simulink model "F90_XMED_02"  (R2025a)
settings: Solver=daessc  StartTime=0.0  StopTime=6  MaxStep=0.6  RelTol=1e-3  AbsTol=1e-3
InitFcn:
  | assert(evalin('base','exist(''target_map_initial_mmHg'',''var'')')==1,'F90:XMED02:MissingPublicInput','Missing target_map_initial_mmHg.');assert(evalin('base','exist(''target_map_final_mmHg'',''var'')')==1,'F90:XMED02:MissingPublicInput','Missing target_map_final_mmHg.');assert(evalin('base','exist(''target_step_time_s'',''var'')')==1,'F90:XMED02:MissingPublicInput','Missing target_step_time_s.');assert(evalin('base','exist(''systemic_resistance_scale'',''var'')')==1,'F90:XMED02:MissingPublicInput','Missing systemic_resistance_scale.');assert(evalin('base','exist(''heart_rate_bpm'',''var'')')==1,'F90:XMED02:MissingPublicInput','Missing heart_rate_bpm.');assert(evalin('base','exist(''pump_speed_limit_rpm'',''var'')')==1,'F90:XMED02:MissingPublicInput','Missing pump_speed_limit_rpm.');f90_mw=get_param(bdroot,'ModelWorkspace');f90_hr=evalin('base','heart_rate_bpm');assignin(f90_mw,'tc',1/(f90_hr/60));assignin(f90_mw,'ts',0.16+0.3/(f90_hr/60));assignin(f90_mw,'R3',evalin('base','systemic_resistance_scale'));assignin(f90_mw,'Tend',6);clear f90_mw f90_hr;
model workspace (MAT data in the model file):
  C1 = 0.22
  C2 = 1.46
  C3 = 20
  C4 = 0.09
  C5 = 2.67
  C6 = 46.7
  EdL = 0.1
  EdR = 0.03
  EsL = 1.375
  EsR = 0.328
  FwVolt = 1e-05
  L1 = 0.000825
  L2 = 0.0036
  L3 = 0.00075
  L4 = 0.00308
  OffCond = 1000
  PipL = 50
  PipR = 24
  R1 = 0.0037511
  R2 = 0.067501
  R3 = 1
  R3_fix = 1
  R3_nominal = 1
  R4 = 0.003751
  R5 = 0.003751
  R6 = 0.03376
  R7 = 0.101
  R8 = 0.003751
  RL = 0.08
  RPM_Setting = 0
  RR = 0.0175
  RmL = 0.08
  RmR = 0.0175
  SetHartRate = 155
  Tend = 6
  WaitTime = 0.022
  X10 = 71.112
  X100 = 23.836
  X110 = 11.294
  X120 = 112.76
  X20 = 8.88
  X30 = 70.516
  X40 = 67.337
  X50 = 3.328
  X60 = 105.52
  X70 = 13.417
  X80 = 0.786
  X90 = 13.393
  capSerRes = 1e-09
  onRes = 0.0001
  tc = 0.8
  ts = 0.4
undefined symbols (not defined in the file): heart_rate_bpm, pump_speed_limit_rpm, systemic_resistance_scale, target_map_final_mmHg, target_map_initial_mmHg, target_step_time_s
libraries: fl_lib x68, nesl_utility x26, ee_lib x4, SignalEditorBlockLib x1
settings Model: Creator=mnord  LastModifiedBy=SimuVerity Contributors
settings SolverCC: ZeroCrossAlgorithm=Adaptive  AlgebraicLoopSolver=TrustRegion
settings DataIOCC: SignalLogging=off
settings DebuggingCC: MaxConsecutiveZCsMsg=warning  IgnoredZcDiagnostic=none  UnconnectedInputMsg=warning  UnconnectedOutputMsg=warning  UnconnectedLineMsg=warning  SymbolicDimsDataTypeCodeGenerationDiagnostic=none
settings ModelReferenceCC: EnableRefExpFcnMdlSchedulingChecks=on
settings SFSimCC: CustomCodeUndefinedFunction=UseInterfaceOnly
settings RTWCC: GPUComputeCapability=3.5  DLArmComputeVersion=19.05
settings SimscapeCC: SimscapeLogSimulationStatistics=on  SimscapeLogDataHistory=10000.0

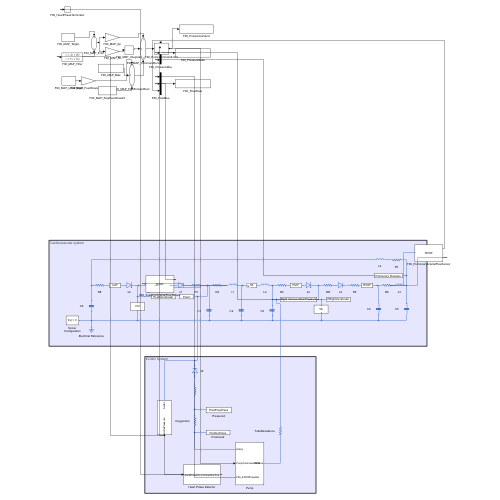
[thumbnail: Simulink's stored preview of the top-level diagram]
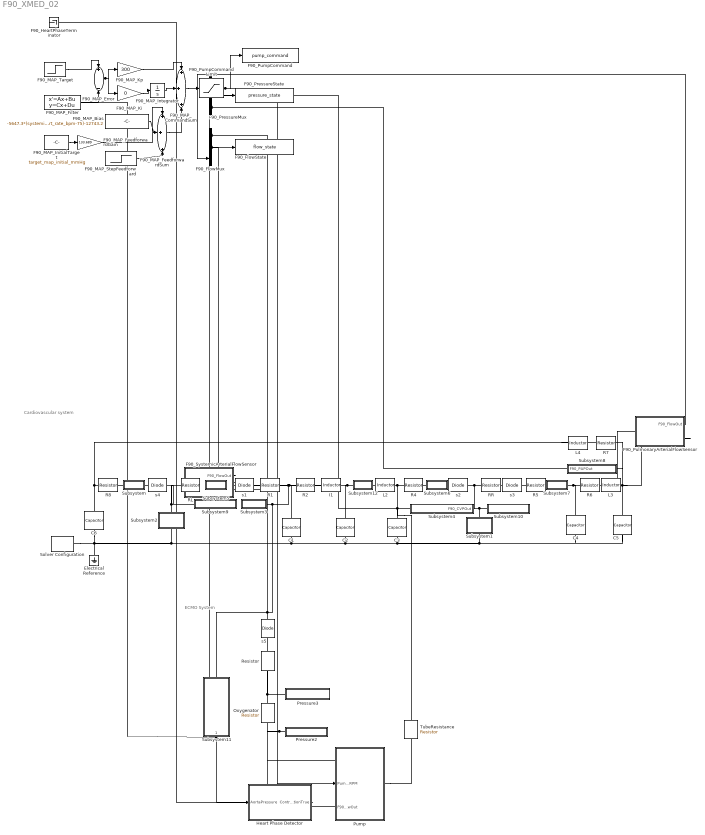
== system F90_XMED_02 ==
  note: Cardiovascular system
  note: ECMO System
  C1 : fl_lib/Electrical/Electrical Elements/Capacitor  c=C1 F  r=capSerRes Ohm  g=0 1/Ohm  i_specify=off  i_priority=None  i=0 A  i_nominal_specify=off  i_nominal_value=1  i_nominal_unit=A  v_specify=off  v_priority=High  v=X10 V  v_nominal_specify=off  v_nominal_value=1  v_nominal_unit=V  vc_specify=on  vc_priority=High  vc=X10 V  vc_nominal_specify=off  vc_nominal_value=1  vc_nominal_unit=V
  C2 : fl_lib/Electrical/Electrical Elements/Capacitor  c=C2 F  r=capSerRes Ohm  g=0 1/Ohm  i_specify=off  i_priority=None  i=0 A  i_nominal_specify=off  i_nominal_value=1  i_nominal_unit=A  v_specify=off  v_priority=High  v=X30 V  v_nominal_specify=off  v_nominal_value=1  v_nominal_unit=V  vc_specify=on  vc_priority=High  vc=X30 V  vc_nominal_specify=off  vc_nominal_value=1  vc_nominal_unit=V
  C3 : fl_lib/Electrical/Electrical Elements/Capacitor  c=C3 F  r=capSerRes Ohm  g=0 1/Ohm  i_specify=off  i_priority=None  i=0 A  i_nominal_specify=off  i_nominal_value=1  i_nominal_unit=A  v_specify=off  v_priority=High  v=X50 V  v_nominal_specify=off  v_nominal_value=1  v_nominal_unit=V  vc_specify=on  vc_priority=High  vc=X50 V  vc_nominal_specify=off  vc_nominal_value=1  vc_nominal_unit=V
  C4 : fl_lib/Electrical/Electrical Elements/Capacitor  c=C4 F  r=capSerRes Ohm  g=0 1/Ohm  i_specify=off  i_priority=None  i=0 A  i_nominal_specify=off  i_nominal_value=1  i_nominal_unit=A  v_specify=off  v_priority=High  v=X70 V  v_nominal_specify=off  v_nominal_value=1  v_nominal_unit=V  vc_specify=on  vc_priority=High  vc=X70 V  vc_nominal_specify=off  vc_nominal_value=1  vc_nominal_unit=V
  C5 : fl_lib/Electrical/Electrical Elements/Capacitor  c=C5 F  r=capSerRes Ohm  g=0 1/Ohm  i_specify=off  i_priority=None  i=0 A  i_nominal_specify=off  i_nominal_value=1  i_nominal_unit=A  v_specify=off  v_priority=High  v=X90 V  v_nominal_specify=off  v_nominal_value=1  v_nominal_unit=V  vc_specify=on  vc_priority=High  vc=X90 V  vc_nominal_specify=off  vc_nominal_value=1  vc_nominal_unit=V
  C6 : fl_lib/Electrical/Electrical Elements/Capacitor  c=C6 F  r=capSerRes Ohm  g=0 1/Ohm  i_specify=off  i_priority=None  i=0 A  i_nominal_specify=off  i_nominal_value=1  i_nominal_unit=A  v_specify=off  v_priority=High  v=X110 V  v_nominal_specify=off  v_nominal_value=1  v_nominal_unit=V  vc_specify=on  vc_priority=High  vc=X110 V  vc_nominal_specify=off  vc_nominal_value=1  vc_nominal_unit=V
  Electrical Reference : fl_lib/Electrical/Electrical Elements/Electrical Reference
  F90_FlowMux : Mux  Inputs=3
  F90_FlowState : ToWorkspace  VariableName=flow_state  SaveFormat=Timeseries  SampleTime=-1
  F90_HeartPhaseTerminator : Terminator
  F90_MAP_Bias : Constant  Value=-5647.3*(systemic_resistance_scale-1)-6.178*(heart_rate_bpm-75)-12743.2
  F90_MAP_CommandSum : Sum  Inputs=+++
  F90_MAP_Error : Sum  Inputs=+-
  F90_MAP_FeedforwardGain : Gain  Gain=133.689
  F90_MAP_FeedforwardSum : Sum  Inputs=+++
  F90_MAP_Filter : StateSpace  A=-1/0.35  B=1/0.35  D=0  InitialCondition=target_map_initial_mmHg
  F90_MAP_InitialTarget : Constant  Value=target_map_initial_mmHg
  F90_MAP_Integrator : Integrator
  F90_MAP_Ki : Gain  Gain=0
  F90_MAP_Kp : Gain  Gain=300
  F90_MAP_StepFeedforward : Step  Time=target_step_time_s  After=90*(target_map_final_mmHg-target_map_initial_mmHg)  SampleTime=0
  F90_MAP_Target : Step  Time=target_step_time_s  Before=target_map_initial_mmHg  After=target_map_final_mmHg  SampleTime=0
  F90_PressureMux : Mux  Inputs=3
  F90_PressureState : ToWorkspace  VariableName=pressure_state  SaveFormat=Timeseries  SampleTime=-1
  F90_PulmonaryArterialFlowSensor : Subsystem
      mask Display: disp('RVOF')
  F90_PumpCommand : ToWorkspace  VariableName=pump_command  SaveFormat=Timeseries  SampleTime=-1
  F90_PumpCommandLimit : Saturate  UpperLimit=pump_speed_limit_rpm  LowerLimit=0
  F90_SystemicArterialFlowSensor : Subsystem
      mask Display: disp('RVOF')
  Heart Phase Detector : Subsystem
  I1 : ee_lib/Passive/Inductor  l=L1 H  enable_L_tol=0  L_tol=20  tol_distribution=1  nSigma=4  r=0 Ohm  g=1e-9 1/Ohm  enable_operating_limits=0  operating_limit_action=2  max_working_current=1 A  power_rating=1 W  i_L_specify=on  i_L_priority=High  i_L=X20 A  i_L_nominal_specify=off  i_L_nominal_value=1  i_L_nominal_unit=A
  L2 : ee_lib/Passive/Inductor  l=L2 H  enable_L_tol=0  L_tol=20  tol_distribution=1  nSigma=4  r=0 Ohm  g=1e-9 1/Ohm  enable_operating_limits=0  operating_limit_action=2  max_working_current=1 A  power_rating=1 W  i_L_specify=on  i_L_priority=High  i_L=X40 A  i_L_nominal_specify=off  i_L_nominal_value=1  i_L_nominal_unit=A
  L3 : ee_lib/Passive/Inductor  l=L3 H  enable_L_tol=0  L_tol=20  tol_distribution=1  nSigma=4  r=0 Ohm  g=1e-9 1/Ohm  enable_operating_limits=0  operating_limit_action=2  max_working_current=1 A  power_rating=1 W  i_L_specify=on  i_L_priority=High  i_L=X80 A  i_L_nominal_specify=off  i_L_nominal_value=1  i_L_nominal_unit=A
  L4 : ee_lib/Passive/Inductor  l=L4 H  enable_L_tol=0  L_tol=20  tol_distribution=1  nSigma=4  r=0 Ohm  g=1e-9 1/Ohm  enable_operating_limits=0  operating_limit_action=2  max_working_current=1 A  power_rating=1 W  i_L_specify=on  i_L_priority=High  i_L=X100 A  i_L_nominal_specify=off  i_L_nominal_value=1  i_L_nominal_unit=A
  Oxygenator : fl_lib/Electrical/Electrical Elements/Resistor  R=1/1.13 Ohm  i_specify=off  i_priority=None  i=0 A  i_nominal_specify=off  i_nominal_value=1  i_nominal_unit=A  v_specify=off  v_priority=None  v=0 V  v_nominal_specify=off  v_nominal_value=1  v_nominal_unit=V
  Pressure2 : Subsystem
      mask Display: disp('PreOxyPress')
  Pressure3 : Subsystem
      mask Display: disp('PostPoxyPress')
  Pump : Subsystem
      settings: PortSchema="{\"entries\":[{\"content\":{\"sides\":[{\"content\":{\"connectorIds\":[\"LConn1\"]},\"type\":\"ConnectorPlacement.EquallySpacedRectSide\",\"uuid\":\"62db16dc-542a-4803-9c2c-9a470fc91885\"},{\"content\":{\"connectorIds\":[\"RConn1\",\"In1\",\"Out1\"],\"side\":\"RIGHT\"},\"type\":\"ConnectorPlacement.EquallySpacedRectSide\",\"uuid\":\"05a4665e-1cd6-4c93-95ba-f78495d840a1\"},{\"content\":{\"side\":\"TOP\"},\"type\":\"ConnectorPlacement.EquallySpacedRectSide\",\"uuid\":\"174192fa-e994-4b45-8a1f-dd44ebe2b866\"},{\"content\":{\"side\":\"BOTTOM\"},\"type\":\"ConnectorPlacement.EquallySpacedRectSide\",\"uuid\":\"194a326f-2a13-4189-b0b8-d4f935dc1fe6\"}]},\"type\":\"ConnectorPlacement.EquallySpacedConnector\",\"uuid\":\"9d7b36c7-1763-48ea-a53e-009c812e3b66\"}],\"packageUris\":[\"http://schema.mathworks.com/mf0/Connector/R2020b\"],\"version\":\"1.0\"}"
  R1 : fl_lib/Electrical/Electrical Elements/Resistor  R=R1 Ohm  i_specify=off  i_priority=None  i=0 A  i_nominal_specify=off  i_nominal_value=1  i_nominal_unit=A  v_specify=off  v_priority=None  v=0 V  v_nominal_specify=off  v_nominal_value=1  v_nominal_unit=V
  R2 : fl_lib/Electrical/Electrical Elements/Resistor  R=R2 Ohm  i_specify=off  i_priority=None  i=0 A  i_nominal_specify=off  i_nominal_value=1  i_nominal_unit=A  v_specify=off  v_priority=None  v=0 V  v_nominal_specify=off  v_nominal_value=1  v_nominal_unit=V
  R4 : fl_lib/Electrical/Electrical Elements/Resistor  R=R4 Ohm  i_specify=off  i_priority=None  i=0 A  i_nominal_specify=off  i_nominal_value=1  i_nominal_unit=A  v_specify=off  v_priority=None  v=0 V  v_nominal_specify=off  v_nominal_value=1  v_nominal_unit=V
  R5 : fl_lib/Electrical/Electrical Elements/Resistor  R=R5 Ohm  i_specify=off  i_priority=None  i=0 A  i_nominal_specify=off  i_nominal_value=1  i_nominal_unit=A  v_specify=off  v_priority=None  v=0 V  v_nominal_specify=off  v_nominal_value=1  v_nominal_unit=V
  R6 : fl_lib/Electrical/Electrical Elements/Resistor  R=R6 Ohm  i_specify=off  i_priority=None  i=0 A  i_nominal_specify=off  i_nominal_value=1  i_nominal_unit=A  v_specify=off  v_priority=None  v=0 V  v_nominal_specify=off  v_nominal_value=1  v_nominal_unit=V
  R7 : fl_lib/Electrical/Electrical Elements/Resistor  R=R7 Ohm  i_specify=off  i_priority=None  i=0 A  i_nominal_specify=off  i_nominal_value=1  i_nominal_unit=A  v_specify=off  v_priority=None  v=0 V  v_nominal_specify=off  v_nominal_value=1  v_nominal_unit=V
  R8 : fl_lib/Electrical/Electrical Elements/Resistor  R=R8 Ohm  i_specify=off  i_priority=None  i=0 A  i_nominal_specify=off  i_nominal_value=1  i_nominal_unit=A  v_specify=off  v_priority=None  v=0 V  v_nominal_specify=off  v_nominal_value=1  v_nominal_unit=V
  RL : fl_lib/Electrical/Electrical Elements/Resistor  R=RL Ohm  i_specify=off  i_priority=None  i=0 A  i_nominal_specify=off  i_nominal_value=1  i_nominal_unit=A  v_specify=off  v_priority=None  v=0 V  v_nominal_specify=off  v_nominal_value=1  v_nominal_unit=V
  RR : fl_lib/Electrical/Electrical Elements/Resistor  R=RR Ohm  i_specify=off  i_priority=None  i=0 A  i_nominal_specify=off  i_nominal_value=1  i_nominal_unit=A  v_specify=off  v_priority=None  v=0 V  v_nominal_specify=off  v_nominal_value=1  v_nominal_unit=V
  Resistor : fl_lib/Electrical/Electrical Elements/Resistor  R=1/1.6 Ohm  i_specify=off  i_priority=None  i=0 A  i_nominal_specify=off  i_nominal_value=1  i_nominal_unit=A  v_specify=off  v_priority=None  v=0 V  v_nominal_specify=off  v_nominal_value=1  v_nominal_unit=V
  Solver Configuration : nesl_utility/Solver Configuration  PhysicalDomain=network_engine_domain  SubClassName=solver  LeftPortType=input  RightPortType=generic  Tones=[]  Harmonics=[]  SimulateNoise=off  Profile=off  UseLocalSampling=off  EnableSwitchedLinearOptims=on  FrequencyDomain=off  UseCCode=off  RelTol=0.001  AbsTol=1e-06  MinStep=1e-09  ToWorkspace=off  RevertToSquareIcSolve=off  NumHomotopyIterations=100  PhasorMode=off  PhasorModeNumHarmonics=1  ConsistencySolver=NEWTON_FTOL  IndexReductionMethod=DerivativeReplacement  DoDC=off  ResidualTolerance=1e-09  ConsistencyTolSource=GLOBAL  ConsistencyAbsTol=0.001  ConsistencyRelTol=0.001  ConsistencyTolFactor=0.001  UseLocalSolver=off  LocalSolverChoice=NE_BACKWARD_EULER_ADVANCER  ResolveIndetEquations=on  FunctionEvalNumThread=1  LocalSolverSampleTime=0.001  DoFixedCost=off  MaxNonlinIter=3  MaxModeIter=2  ComputeImpulses=off  ImpulseIterations=2  LinearAlgebra=auto  LinearAlgebraNumThread=0  EquationFormulation=NE_TIME_EF  DelaysMemoryBudget=1024  AutomaticFiltering=on  FilteringTimeConstant=0.001  PartitionStorageMethod=AS_NEEDED  PartitionMemoryBudget=1024  PartitionMethod=ROBUST  MultibodyUseLocalSolver=off  MultibodyLocalSolverChoice=ODE1  MultibodyLocalSolverSampleTime=0.001
  Subsystem : Subsystem
      mask Display: disp('LVIF')
  Subsystem1 : Subsystem
      mask Display: disp('V6')
  Subsystem10 : Subsystem
      mask Display: disp('PRightVentricular')
  Subsystem11 : Subsystem
      settings: PortSchema="{\"entries\":[{\"content\":{\"sides\":[{\"content\":{\"connectorIds\":[]},\"type\":\"ConnectorPlacement.EquallySpacedRectSide\",\"uuid\":\"f9ffc3b3-0f3f-4df5-be7e-a65199d8fb18\"},{\"content\":{\"connectorIds\":[],\"side\":\"RIGHT\"},\"type\":\"ConnectorPlacement.EquallySpacedRectSide\",\"uuid\":\"6b3c46a3-b656-482e-b0a9-93777308e083\"},{\"content\":{\"connectorIds\":[\"LConn1\"],\"side\":\"TOP\"},\"type\":\"ConnectorPlacement.EquallySpacedRectSide\",\"uuid\":\"e2309b6a-a528-4e82-8df5-2fdb2444f40a\"},{\"content\":{\"connectorIds\":[\"Out1\"],\"side\":\"BOTTOM\"},\"type\":\"ConnectorPlacement.EquallySpacedRectSide\",\"uuid\":\"7e89f23f-224f-485d-9e96-fb39bd2403a7\"}]},\"type\":\"ConnectorPlacement.EquallySpacedConnector\",\"uuid\":\"798f20cf-0f77-4082-bc02-f5f2bf5391c0\"}],\"packageUris\":[\"http://schema.mathworks.com/mf0/Connector/R2020b\"],\"version\":\"1.0\"}"
  Subsystem12 : Subsystem  Variant=on  VariantControlMode=label  VariantControl=Choice  LabelModeActiveChoice=R3_Fix
      mask Display: disp('R3')
  Subsystem2 : Subsystem
      mask Display: disp('V12')
  Subsystem3 : Subsystem
      mask Display: disp('Paort')
  Subsystem4 : Subsystem
      mask Display: disp('Right Venous Atrial Pressure')
  Subsystem5 : Subsystem
      mask Display: disp('LVOF')
  Subsystem6 : Subsystem
      mask Display: disp('RVIF')
  Subsystem7 : Subsystem
      mask Display: disp('RVOF')
  Subsystem8 : Subsystem
      mask Display: disp('Pulmonary Pressure')
  Subsystem9 : Subsystem
      mask Display: disp('PLeftVentricular')
  TubeResistance : fl_lib/Electrical/Electrical Elements/Resistor  R=1 Ohm  i_specify=off  i_priority=None  i=60 A  i_nominal_specify=off  i_nominal_value=1  i_nominal_unit=A  v_specify=off  v_priority=None  v=0 V  v_nominal_specify=off  v_nominal_value=1  v_nominal_unit=V
  s{1..4} (4 alike) : fl_lib/Electrical/Electrical Elements/Diode  Vf=FwVolt V  Ron=onRes Ohm  Goff=1e-8 1/Ohm  i_specify=off  i_priority=None  i=0 A  i_nominal_specify=off  i_nominal_value=1  i_nominal_unit=A  v_specify=off  v_priority=None  v=0 V  v_nominal_specify=off  v_nominal_value=1  v_nominal_unit=V
  s5 : fl_lib/Electrical/Electrical Elements/Diode  Vf=FwVolt V  Ron=0.54*0.1 Ohm  Goff=1e-8 1/Ohm  i_specify=off  i_priority=None  i=0 A  i_nominal_specify=off  i_nominal_value=1  i_nominal_unit=A  v_specify=off  v_priority=None  v=0 V  v_nominal_specify=off  v_nominal_value=1  v_nominal_unit=V
  wires:
  Subsystem11/1(AortaPressure) -> Heart Phase Detector/1(AortaPressure), F90_PressureMux/1, F90_MAP_Filter/1
  Heart Phase Detector/1(ContractionTrue) -> F90_HeartPhaseTerminator/1
  Subsystem4/1(F90_CVPOut) -> F90_PressureMux/2
  Subsystem8/1(F90_PAPOut) -> F90_PressureMux/3
  F90_PressureMux/1 -> F90_PressureState/1
  Pump/1(F90_ECMOFlowOut) -> F90_FlowMux/1
  F90_SystemicArterialFlowSensor/1(F90_FlowOut) -> F90_FlowMux/2
  F90_PulmonaryArterialFlowSensor/1(F90_FlowOut) -> F90_FlowMux/3
  F90_FlowMux/1 -> F90_FlowState/1
  F90_MAP_Target/1 -> F90_MAP_Error/1
  F90_MAP_Filter/1 -> F90_MAP_Error/2
  F90_MAP_Error/1 -> F90_MAP_Kp/1, F90_MAP_Ki/1
  F90_MAP_Kp/1 -> F90_MAP_CommandSum/1
  F90_MAP_Ki/1 -> F90_MAP_Integrator/1
  F90_MAP_Integrator/1 -> F90_MAP_CommandSum/2
  F90_MAP_InitialTarget/1 -> F90_MAP_FeedforwardGain/1
  F90_MAP_FeedforwardGain/1 -> F90_MAP_FeedforwardSum/1
  F90_MAP_Bias/1 -> F90_MAP_FeedforwardSum/2
  F90_MAP_StepFeedforward/1 -> F90_MAP_FeedforwardSum/3
  F90_MAP_FeedforwardSum/1 -> F90_MAP_CommandSum/3
  F90_MAP_CommandSum/1 -> F90_PumpCommandLimit/1
  F90_PumpCommandLimit/1 -> Pump/1(PumpCommandRPM), F90_PumpCommand/1
  connections:
  s1/LConn1 -- Subsystem5/RConn1
  s2/LConn1 -- Subsystem6/RConn1
  R5/RConn1 -- Subsystem7/LConn1
  s4/LConn1 -- Subsystem/RConn1
  R6/LConn1 -- C4/LConn1 -- Subsystem7/RConn1
  Subsystem12/RConn1 -- L2/LConn1
  Subsystem5/LConn1 -- RL/RConn1
  L3/RConn1 -- Subsystem8/LConn1 -- R7/LConn1 -- C5/LConn1
  Subsystem6/LConn1 -- R4/RConn1
  C6/LConn1 -- R8/LConn1 -- L4/RConn1
  s1/RConn1 -- R1/LConn1
  s3/RConn1 -- R5/LConn1
  R7/RConn1 -- L4/LConn1
  R8/RConn1 -- Subsystem/LConn1
  Subsystem10/LConn1 -- Subsystem1/LConn1 -- RR/LConn1 -- s2/RConn1
  s4/RConn1 -- RL/LConn1 -- Subsystem9/LConn1 -- Subsystem2/LConn1
  s3/LConn1 -- RR/RConn1
  C6/RConn1 -- Electrical Reference/LConn1 -- C5/RConn1 -- C4/RConn1 -- Subsystem1/RConn1 -- C3/RConn1 -- C2/RConn1 -- C1/RConn1 -- Subsystem2/RConn1 -- Solver Configuration/RConn1
  I1/RConn1 -- C2/LConn1 -- Subsystem12/LConn1
  Pressure2/RConn1 -- Pump/RConn1 -- Oxygenator/LConn1
  R4/LConn1 -- TubeResistance/LConn1 -- Subsystem4/LConn1 -- C3/LConn1 -- L2/RConn1
  Resistor/RConn1 -- s5/LConn1
  Oxygenator/RConn1 -- Resistor/LConn1 -- Pressure3/RConn1
  Pump/LConn1 -- TubeResistance/RConn1
  C1/LConn1 -- R1/RConn1 -- Subsystem11/LConn1 -- s5/RConn1 -- Subsystem3/LConn1 -- R2/LConn1
  R2/RConn1 -- F90_SystemicArterialFlowSensor/LConn1
  F90_SystemicArterialFlowSensor/RConn1 -- I1/LConn1
  R6/RConn1 -- F90_PulmonaryArterialFlowSensor/LConn1
  F90_PulmonaryArterialFlowSensor/RConn1 -- L3/LConn1

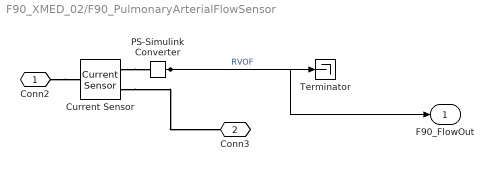
== system F90_XMED_02/F90_PulmonaryArterialFlowSensor ==
  Current Sensor : fl_lib/Electrical/Electrical Sensors/Current Sensor
  PS-Simulink Converter : nesl_utility/PS-Simulink Converter  PhysicalDomain=network_engine_domain  SubClassName=ps_output  LeftPortType=input  RightPortType=output  PseudoPeriodic=off  Frequencies=[]  VectorFormat=1-D array  Unit=inherit  AffineConversion=off
  Terminator : Terminator
  Conn2 : PMIOPort  Side=Left
  Conn3 : PMIOPort  Port=2  Side=Right
  F90_FlowOut : Outport
  wires:
  PS-Simulink Converter/1 -> Terminator/1, F90_FlowOut/1  "RVOF"
  connections:
  Current Sensor/RConn1 -- PS-Simulink Converter/LConn1
  Current Sensor/RConn2 -- Conn3/RConn1
  Conn2/RConn1 -- Current Sensor/LConn1

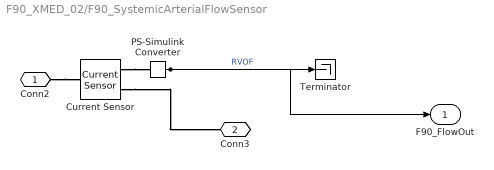
== system F90_XMED_02/F90_SystemicArterialFlowSensor ==
  Current Sensor : fl_lib/Electrical/Electrical Sensors/Current Sensor
  PS-Simulink Converter : nesl_utility/PS-Simulink Converter  PhysicalDomain=network_engine_domain  SubClassName=ps_output  LeftPortType=input  RightPortType=output  PseudoPeriodic=off  Frequencies=[]  VectorFormat=1-D array  Unit=inherit  AffineConversion=off
  Terminator : Terminator
  Conn2 : PMIOPort  Side=Left
  Conn3 : PMIOPort  Port=2  Side=Right
  F90_FlowOut : Outport
  wires:
  PS-Simulink Converter/1 -> Terminator/1, F90_FlowOut/1  "RVOF"
  connections:
  Current Sensor/RConn1 -- PS-Simulink Converter/LConn1
  Current Sensor/RConn2 -- Conn3/RConn1
  Conn2/RConn1 -- Current Sensor/LConn1

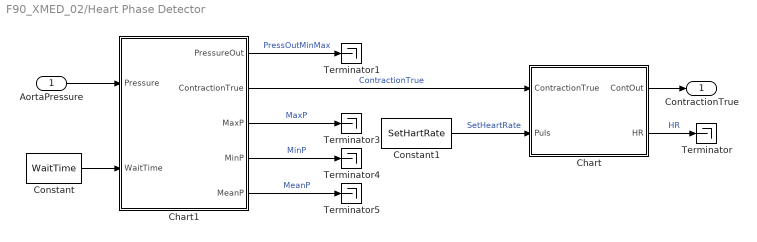
== system F90_XMED_02/Heart Phase Detector ==
  AortaPressure : Inport
  Chart : Stateflow chart  TreatAsAtomicUnit=on
  Chart1 : Stateflow chart  TreatAsAtomicUnit=on
  Constant : Constant  Value=WaitTime
  Constant1 : Constant  Value=SetHartRate
  Terminator{,1,3..5} (5 alike) : Terminator
  ContractionTrue : Outport
  wires:
  AortaPressure/1 -> Chart1/1(Pressure)
  Chart1/1(PressureOut) -> Terminator1/1  "PressOutMinMax"
  Chart1/2(ContractionTrue) -> Chart/1(ContractionTrue)  "ContractionTrue"
  Chart1/4(MinP) -> Terminator4/1  "MinP"
  Chart1/3(MaxP) -> Terminator3/1  "MaxP"
  Chart1/5(MeanP) -> Terminator5/1  "MeanP"
  Constant/1 -> Chart1/2(WaitTime)
  Chart/1(ContOut) -> ContractionTrue/1
  Chart/2(HR) -> Terminator/1  "HR"
  Constant1/1 -> Chart/2(Puls)  "SetHeartRate"

== system F90_XMED_02/Pressure2 ==
  Electrical Reference1 : fl_lib/Electrical/Electrical Elements/Electrical Reference
  Pre Oxy P2 : nesl_utility/PS-Simulink Converter  PhysicalDomain=network_engine_domain  SubClassName=ps_output  LeftPortType=input  RightPortType=output  PseudoPeriodic=off  Frequencies=[]  VectorFormat=1-D array  Unit=inherit  AffineConversion=off
  Pressure 2 : Scope
      settings: ActiveDisplayYMinimum=-9.53147  ActiveDisplayYMaximum=105.78415
  Voltage Sensor : fl_lib/Electrical/Electrical Sensors/Voltage Sensor
  Conn1 : PMIOPort  Side=Right
  wires:
  Pre Oxy P2/1 -> Pressure 2/1
  connections:
  Voltage Sensor/RConn1 -- Pre Oxy P2/LConn1
  Voltage Sensor/LConn1 -- Conn1/RConn1
  Voltage Sensor/RConn2 -- Electrical Reference1/LConn1

== system F90_XMED_02/Pressure3 ==
  Electrical Reference2 : fl_lib/Electrical/Electrical Elements/Electrical Reference
  Post Oxy P3 : nesl_utility/PS-Simulink Converter  PhysicalDomain=network_engine_domain  SubClassName=ps_output  LeftPortType=input  RightPortType=output  PseudoPeriodic=off  Frequencies=[]  VectorFormat=1-D array  Unit=inherit  AffineConversion=off
  Pressure3 : Scope
      settings: ActiveDisplayYMinimum=74.08538  ActiveDisplayYMaximum=102.93086
  Voltage Sensor : fl_lib/Electrical/Electrical Sensors/Voltage Sensor
  Conn1 : PMIOPort  Side=Right
  wires:
  Post Oxy P3/1 -> Pressure3/1
  connections:
  Voltage Sensor/RConn1 -- Post Oxy P3/LConn1
  Electrical Reference2/LConn1 -- Voltage Sensor/RConn2
  Conn1/RConn1 -- Voltage Sensor/LConn1

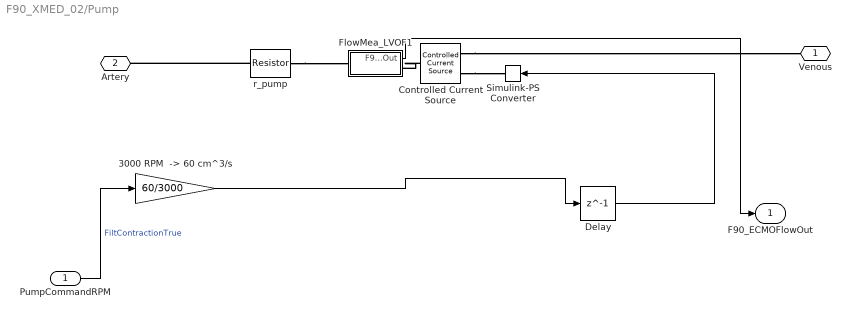
== system F90_XMED_02/Pump ==
  PumpCommandRPM : Inport
  "3000 RPM  -> 60 cm^3/s" : Gain  Gain=60/3000
  Controlled Current Source : fl_lib/Electrical/Electrical Sources/Controlled Current Source
  Delay : Delay  DelayLength=1  SampleTime=0.001
  FlowMea_LVOF1 : Subsystem
      mask Display: disp('EcmoFlow')
  Simulink-PS Converter : nesl_utility/Simulink-PS Converter  PhysicalDomain=network_engine_domain  SubClassName=ps_input  LeftPortType=input  RightPortType=output  PseudoPeriodic=off  Frequencies=[]  NoiseDistribution=none  NoiseParameters=[]  Unit=1  AffineConversion=off  FilteringAndDerivatives=filter  SimscapeFilterOrder=1  InputFilterTimeConstant=0.001  UdotUserProvided=0
  r_pump : fl_lib/Electrical/Electrical Elements/Resistor  R=1/1.68 Ohm  i_specify=on  i_priority=None  i=83.3 A  i_nominal_specify=off  i_nominal_value=1  i_nominal_unit=A  v_specify=off  v_priority=None  v=0 V  v_nominal_specify=off  v_nominal_value=1  v_nominal_unit=V
  Venous : PMIOPort  Side=Left
  Artery : PMIOPort  Port=2  Side=Right
  F90_ECMOFlowOut : Outport
  wires:
  Delay/1 -> Simulink-PS Converter/1
  PumpCommandRPM/1 -> "3000 RPM  -> 60 cm^3/s"/1  "FiltContractionTrue"
  "3000 RPM  -> 60 cm^3/s"/1 -> Delay/1
  FlowMea_LVOF1/1(F90_ECMOFlowOut) -> F90_ECMOFlowOut/1
  connections:
  Controlled Current Source/RConn2 -- Venous/RConn1
  r_pump/LConn1 -- FlowMea_LVOF1/LConn1
  Controlled Current Source/RConn1 -- Simulink-PS Converter/RConn1
  r_pump/RConn1 -- Artery/RConn1
  Controlled Current Source/LConn1 -- FlowMea_LVOF1/RConn1

== system F90_XMED_02/Subsystem ==
  Current Sensor : fl_lib/Electrical/Electrical Sensors/Current Sensor
  PS-Simulink Converter : nesl_utility/PS-Simulink Converter  PhysicalDomain=network_engine_domain  SubClassName=ps_output  LeftPortType=input  RightPortType=output  PseudoPeriodic=off  Frequencies=[]  VectorFormat=1-D array  Unit=inherit  AffineConversion=off
  Terminator : Terminator
  Conn2 : PMIOPort  Side=Left
  Conn3 : PMIOPort  Port=2  Side=Right
  wires:
  PS-Simulink Converter/1 -> Terminator/1  "LVIF"
  connections:
  Conn2/RConn1 -- Current Sensor/LConn1
  Current Sensor/RConn2 -- Conn3/RConn1
  Current Sensor/RConn1 -- PS-Simulink Converter/LConn1

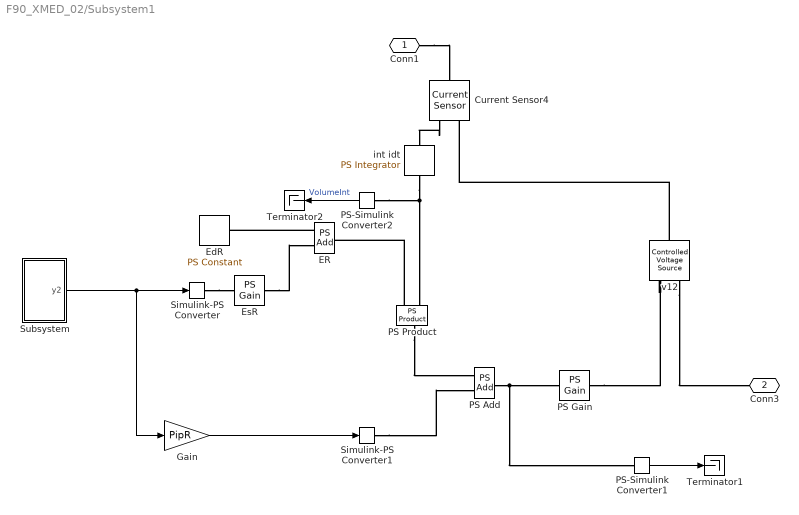
== system F90_XMED_02/Subsystem1 ==
  Current Sensor4 : fl_lib/Electrical/Electrical Sensors/Current Sensor
  ER : fl_lib/Physical Signals/Functions/PS Add
  EdR : fl_lib/Physical Signals/Sources/PS Constant  constant=EdR
  EsR : fl_lib/Physical Signals/Functions/PS Gain  gain=EsR
  Gain : Gain  Gain=PipR
  PS Add : fl_lib/Physical Signals/Functions/PS Add
  PS Gain : fl_lib/Physical Signals/Functions/PS Gain  gain=1 V/s/A
  PS Product : fl_lib/Physical Signals/Functions/PS Product
  PS-Simulink Converter1 : nesl_utility/PS-Simulink Converter  PhysicalDomain=network_engine_domain  SubClassName=ps_output  LeftPortType=input  RightPortType=output  PseudoPeriodic=off  Frequencies=[]  VectorFormat=1-D array  Unit=inherit  AffineConversion=off
  PS-Simulink Converter2 : nesl_utility/PS-Simulink Converter  PhysicalDomain=network_engine_domain  SubClassName=ps_output  LeftPortType=input  RightPortType=output  PseudoPeriodic=off  Frequencies=[]  VectorFormat=1-D array  Unit=inherit  AffineConversion=off
  Simulink-PS Converter : nesl_utility/Simulink-PS Converter  PhysicalDomain=network_engine_domain  SubClassName=ps_input  LeftPortType=input  RightPortType=output  PseudoPeriodic=off  Frequencies=[]  NoiseDistribution=none  NoiseParameters=[]  Unit=1  AffineConversion=off  FilteringAndDerivatives=provide  SimscapeFilterOrder=1  InputFilterTimeConstant=0.001  UdotUserProvided=0
  Simulink-PS Converter1 : nesl_utility/Simulink-PS Converter  PhysicalDomain=network_engine_domain  SubClassName=ps_input  LeftPortType=input  RightPortType=output  PseudoPeriodic=off  Frequencies=[]  NoiseDistribution=none  NoiseParameters=[]  Unit=A*s  AffineConversion=off  FilteringAndDerivatives=provide  SimscapeFilterOrder=1  InputFilterTimeConstant=0.001  UdotUserProvided=0
  Subsystem : Subsystem
  Terminator1 : Terminator
  Terminator2 : Terminator
  int idt : fl_lib/Physical Signals/Linear Operators/PS Integrator  reset_method=foundation.enum.IntegratorResetSpec.None  initial_condition_spec=foundation.enum.IntegratorICSpec.Internal  saturation_spec=foundation.enum.IntegratorSaturationSpec.None  saturation_source_spec=foundation.enum.IntegratorSaturationSourceSpec.Internal  x0=X60 A*s  xu=inf s  xl=-inf s
  v12 : fl_lib/Electrical/Electrical Sources/Controlled Voltage Source
  Conn1 : PMIOPort  Side=Left
  Conn3 : PMIOPort  Port=2  Side=Right
  wires:
  PS-Simulink Converter1/1 -> Terminator1/1
  Gain/1 -> Simulink-PS Converter1/1
  PS-Simulink Converter2/1 -> Terminator2/1  "VolumeInt"
  Subsystem/1(y2) -> Gain/1, Simulink-PS Converter/1
  connections:
  PS Add/RConn1 -- PS-Simulink Converter1/LConn1 -- PS Gain/LConn1
  PS-Simulink Converter2/LConn1 -- PS Product/LConn1 -- int idt/RConn1
  PS Product/RConn1 -- PS Add/LConn1
  v12/LConn1 -- Current Sensor4/RConn2
  ER/LConn1 -- EdR/RConn1
  Simulink-PS Converter1/RConn1 -- PS Add/LConn2
  EsR/RConn1 -- ER/LConn2
  PS Product/LConn2 -- ER/RConn1
  v12/RConn2 -- Conn3/RConn1
  Conn1/RConn1 -- Current Sensor4/LConn1
  Current Sensor4/RConn1 -- int idt/LConn1
  Simulink-PS Converter/RConn1 -- EsR/LConn1
  PS Gain/RConn1 -- v12/RConn1

== system F90_XMED_02/Subsystem10 ==
  Electrical Reference1 : fl_lib/Electrical/Electrical Elements/Electrical Reference
  PS-Simulink Converter : nesl_utility/PS-Simulink Converter  PhysicalDomain=network_engine_domain  SubClassName=ps_output  LeftPortType=input  RightPortType=output  PseudoPeriodic=off  Frequencies=[]  VectorFormat=1-D array  Unit=inherit  AffineConversion=off
  Terminator : Terminator
  Voltage Sensor : fl_lib/Electrical/Electrical Sensors/Voltage Sensor
  Conn1 : PMIOPort  Side=Left
  wires:
  PS-Simulink Converter/1 -> Terminator/1  "Right Ventricular Pressure"
  connections:
  Conn1/RConn1 -- Voltage Sensor/LConn1
  Voltage Sensor/RConn2 -- Electrical Reference1/LConn1
  Voltage Sensor/RConn1 -- PS-Simulink Converter/LConn1

== system F90_XMED_02/Subsystem11 ==
  Electrical Reference : fl_lib/Electrical/Electrical Elements/Electrical Reference
  PS-Simulink Converter : nesl_utility/PS-Simulink Converter  PhysicalDomain=network_engine_domain  SubClassName=ps_output  LeftPortType=input  RightPortType=output  PseudoPeriodic=off  Frequencies=[]  VectorFormat=1-D array  Unit=inherit  AffineConversion=off
  Voltage Sensor : fl_lib/Electrical/Electrical Sensors/Voltage Sensor
  Aorta1 : PMIOPort  Side=Left
  AortaPressure : Outport
  wires:
  PS-Simulink Converter/1 -> AortaPressure/1
  connections:
  Voltage Sensor/LConn1 -- Aorta1/RConn1
  Voltage Sensor/RConn2 -- Electrical Reference/LConn1
  Voltage Sensor/RConn1 -- PS-Simulink Converter/LConn1

== system F90_XMED_02/Subsystem12 ==
  Fixed : Subsystem  VariantControl=R3_Fix
  Variable : Subsystem  VariantControl=R3_Variant
  Conn1 : PMIOPort  Side=Left
  Conn2 : PMIOPort  Port=2  Side=Right

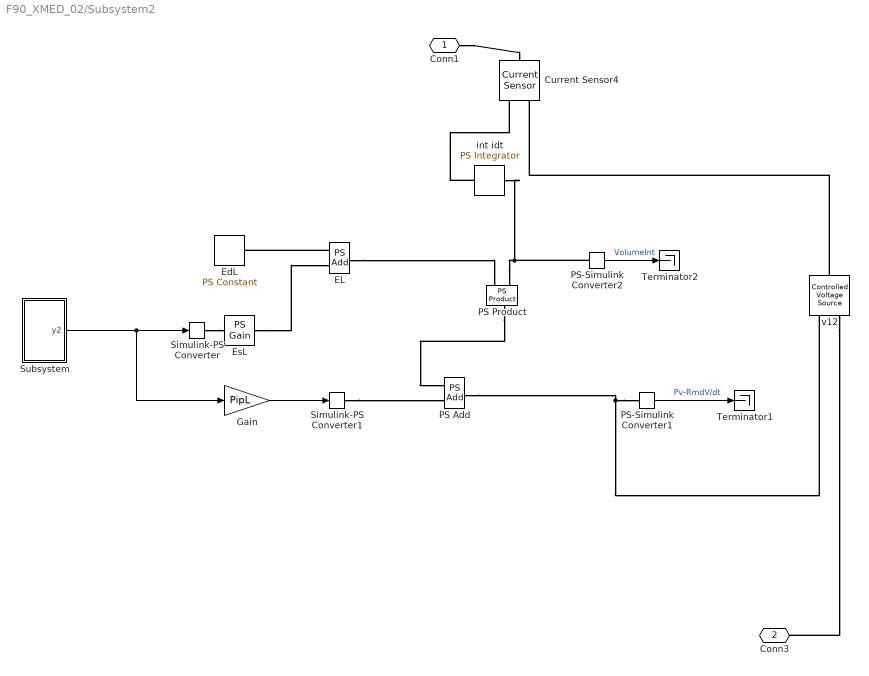
== system F90_XMED_02/Subsystem2 ==
  Current Sensor4 : fl_lib/Electrical/Electrical Sensors/Current Sensor
  EL : fl_lib/Physical Signals/Functions/PS Add
  EdL : fl_lib/Physical Signals/Sources/PS Constant  constant=EdL V/A/s
  EsL : fl_lib/Physical Signals/Functions/PS Gain  gain=EsL
  Gain : Gain  Gain=PipL
  PS Add : fl_lib/Physical Signals/Functions/PS Add
  PS Product : fl_lib/Physical Signals/Functions/PS Product
  PS-Simulink Converter1 : nesl_utility/PS-Simulink Converter  PhysicalDomain=network_engine_domain  SubClassName=ps_output  LeftPortType=input  RightPortType=output  PseudoPeriodic=off  Frequencies=[]  VectorFormat=1-D array  Unit=inherit  AffineConversion=off
  PS-Simulink Converter2 : nesl_utility/PS-Simulink Converter  PhysicalDomain=network_engine_domain  SubClassName=ps_output  LeftPortType=input  RightPortType=output  PseudoPeriodic=off  Frequencies=[]  VectorFormat=1-D array  Unit=inherit  AffineConversion=off
  Simulink-PS Converter : nesl_utility/Simulink-PS Converter  PhysicalDomain=network_engine_domain  SubClassName=ps_input  LeftPortType=input  RightPortType=output  PseudoPeriodic=off  Frequencies=[]  NoiseDistribution=none  NoiseParameters=[]  Unit=V/A/s  AffineConversion=off  FilteringAndDerivatives=provide  SimscapeFilterOrder=1  InputFilterTimeConstant=0.001  UdotUserProvided=0
  Simulink-PS Converter1 : nesl_utility/Simulink-PS Converter  PhysicalDomain=network_engine_domain  SubClassName=ps_input  LeftPortType=input  RightPortType=output  PseudoPeriodic=off  Frequencies=[]  NoiseDistribution=none  NoiseParameters=[]  Unit=V  AffineConversion=off  FilteringAndDerivatives=provide  SimscapeFilterOrder=1  InputFilterTimeConstant=0.001  UdotUserProvided=0
  Subsystem : Subsystem
  Terminator1 : Terminator
  Terminator2 : Terminator
  int idt : fl_lib/Physical Signals/Linear Operators/PS Integrator  reset_method=foundation.enum.IntegratorResetSpec.None  initial_condition_spec=foundation.enum.IntegratorICSpec.Internal  saturation_spec=foundation.enum.IntegratorSaturationSpec.None  saturation_source_spec=foundation.enum.IntegratorSaturationSourceSpec.Internal  x0=X120 A*s  xu=inf s  xl=-inf s
  v12 : fl_lib/Electrical/Electrical Sources/Controlled Voltage Source
  Conn1 : PMIOPort  Side=Left
  Conn3 : PMIOPort  Port=2  Side=Right
  wires:
  Gain/1 -> Simulink-PS Converter1/1
  Subsystem/1(y2) -> Gain/1, Simulink-PS Converter/1
  PS-Simulink Converter1/1 -> Terminator1/1  "Pv-RmdV/dt"
  PS-Simulink Converter2/1 -> Terminator2/1  "VolumeInt"
  connections:
  PS Product/LConn1 -- int idt/RConn1 -- PS-Simulink Converter2/LConn1
  EL/LConn1 -- EdL/RConn1
  PS Product/RConn1 -- PS Add/LConn1
  EsL/RConn1 -- EL/LConn2
  Simulink-PS Converter1/RConn1 -- PS Add/LConn2
  Simulink-PS Converter/RConn1 -- EsL/LConn1
  v12/RConn2 -- Conn3/RConn1
  int idt/LConn1 -- Current Sensor4/RConn1
  Conn1/RConn1 -- Current Sensor4/LConn1
  EL/RConn1 -- PS Product/LConn2
  PS-Simulink Converter1/LConn1 -- PS Add/RConn1 -- v12/RConn1
  v12/LConn1 -- Current Sensor4/RConn2

== system F90_XMED_02/Subsystem3 ==
  Electrical Reference1 : fl_lib/Electrical/Electrical Elements/Electrical Reference
  PS-Simulink Converter : nesl_utility/PS-Simulink Converter  PhysicalDomain=network_engine_domain  SubClassName=ps_output  LeftPortType=input  RightPortType=output  PseudoPeriodic=off  Frequencies=[]  VectorFormat=1-D array  Unit=inherit  AffineConversion=off
  Terminator : Terminator
  Voltage Sensor : fl_lib/Electrical/Electrical Sensors/Voltage Sensor
  Conn1 : PMIOPort  Side=Left
  wires:
  PS-Simulink Converter/1 -> Terminator/1  "Aortic Pressure"
  connections:
  Voltage Sensor/RConn1 -- PS-Simulink Converter/LConn1
  Voltage Sensor/RConn2 -- Electrical Reference1/LConn1
  Conn1/RConn1 -- Voltage Sensor/LConn1

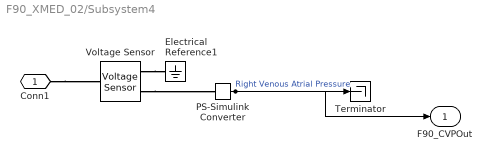
== system F90_XMED_02/Subsystem4 ==
  Electrical Reference1 : fl_lib/Electrical/Electrical Elements/Electrical Reference
  PS-Simulink Converter : nesl_utility/PS-Simulink Converter  PhysicalDomain=network_engine_domain  SubClassName=ps_output  LeftPortType=input  RightPortType=output  PseudoPeriodic=off  Frequencies=[]  VectorFormat=1-D array  Unit=inherit  AffineConversion=off
  Terminator : Terminator
  Voltage Sensor : fl_lib/Electrical/Electrical Sensors/Voltage Sensor
  Conn1 : PMIOPort  Side=Left
  F90_CVPOut : Outport
  wires:
  PS-Simulink Converter/1 -> Terminator/1, F90_CVPOut/1  "Right Venous Atrial Pressure"
  connections:
  Conn1/RConn1 -- Voltage Sensor/LConn1
  Voltage Sensor/RConn2 -- Electrical Reference1/LConn1
  Voltage Sensor/RConn1 -- PS-Simulink Converter/LConn1

== system F90_XMED_02/Subsystem5 ==
  Current Sensor : fl_lib/Electrical/Electrical Sensors/Current Sensor
  PS-Simulink Converter : nesl_utility/PS-Simulink Converter  PhysicalDomain=network_engine_domain  SubClassName=ps_output  LeftPortType=input  RightPortType=output  PseudoPeriodic=off  Frequencies=[]  VectorFormat=1-D array  Unit=inherit  AffineConversion=off
  Terminator : Terminator
  Conn2 : PMIOPort  Side=Left
  Conn3 : PMIOPort  Port=2  Side=Right
  wires:
  PS-Simulink Converter/1 -> Terminator/1  "LVOF"
  connections:
  Conn2/RConn1 -- Current Sensor/LConn1
  Current Sensor/RConn2 -- Conn3/RConn1
  Current Sensor/RConn1 -- PS-Simulink Converter/LConn1

== system F90_XMED_02/Subsystem6 ==
  Current Sensor : fl_lib/Electrical/Electrical Sensors/Current Sensor
  PS-Simulink Converter : nesl_utility/PS-Simulink Converter  PhysicalDomain=network_engine_domain  SubClassName=ps_output  LeftPortType=input  RightPortType=output  PseudoPeriodic=off  Frequencies=[]  VectorFormat=1-D array  Unit=inherit  AffineConversion=off
  Terminator : Terminator
  Conn2 : PMIOPort  Side=Left
  Conn3 : PMIOPort  Port=2  Side=Right
  wires:
  PS-Simulink Converter/1 -> Terminator/1  "RVIF"
  connections:
  Current Sensor/RConn1 -- PS-Simulink Converter/LConn1
  Current Sensor/RConn2 -- Conn3/RConn1
  Conn2/RConn1 -- Current Sensor/LConn1

== system F90_XMED_02/Subsystem7 ==
  Current Sensor : fl_lib/Electrical/Electrical Sensors/Current Sensor
  PS-Simulink Converter : nesl_utility/PS-Simulink Converter  PhysicalDomain=network_engine_domain  SubClassName=ps_output  LeftPortType=input  RightPortType=output  PseudoPeriodic=off  Frequencies=[]  VectorFormat=1-D array  Unit=inherit  AffineConversion=off
  Terminator : Terminator
  Conn2 : PMIOPort  Side=Left
  Conn3 : PMIOPort  Port=2  Side=Right
  wires:
  PS-Simulink Converter/1 -> Terminator/1  "RVOF"
  connections:
  Conn2/RConn1 -- Current Sensor/LConn1
  Current Sensor/RConn2 -- Conn3/RConn1
  Current Sensor/RConn1 -- PS-Simulink Converter/LConn1

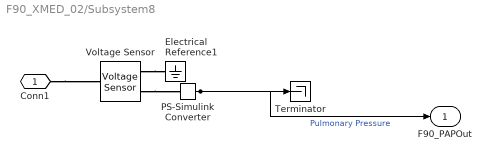
== system F90_XMED_02/Subsystem8 ==
  Electrical Reference1 : fl_lib/Electrical/Electrical Elements/Electrical Reference
  PS-Simulink Converter : nesl_utility/PS-Simulink Converter  PhysicalDomain=network_engine_domain  SubClassName=ps_output  LeftPortType=input  RightPortType=output  PseudoPeriodic=off  Frequencies=[]  VectorFormat=1-D array  Unit=inherit  AffineConversion=off
  Terminator : Terminator
  Voltage Sensor : fl_lib/Electrical/Electrical Sensors/Voltage Sensor
  Conn1 : PMIOPort  Side=Left
  F90_PAPOut : Outport
  wires:
  PS-Simulink Converter/1 -> Terminator/1, F90_PAPOut/1  "Pulmonary Pressure"
  connections:
  Conn1/RConn1 -- Voltage Sensor/LConn1
  Voltage Sensor/RConn2 -- Electrical Reference1/LConn1
  Voltage Sensor/RConn1 -- PS-Simulink Converter/LConn1

== system F90_XMED_02/Subsystem9 ==
  Electrical Reference1 : fl_lib/Electrical/Electrical Elements/Electrical Reference
  PS-Simulink Converter : nesl_utility/PS-Simulink Converter  PhysicalDomain=network_engine_domain  SubClassName=ps_output  LeftPortType=input  RightPortType=output  PseudoPeriodic=off  Frequencies=[]  VectorFormat=1-D array  Unit=inherit  AffineConversion=off
  Terminator : Terminator
  Voltage Sensor : fl_lib/Electrical/Electrical Sensors/Voltage Sensor
  Conn1 : PMIOPort  Side=Left
  wires:
  PS-Simulink Converter/1 -> Terminator/1  "Left Ventricular Pressure"
  connections:
  Conn1/RConn1 -- Voltage Sensor/LConn1
  Voltage Sensor/RConn2 -- Electrical Reference1/LConn1
  Voltage Sensor/RConn1 -- PS-Simulink Converter/LConn1

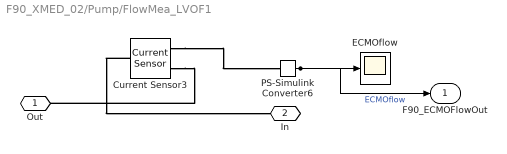
== system F90_XMED_02/Pump/FlowMea_LVOF1 ==
  Current Sensor3 : fl_lib/Electrical/Electrical Sensors/Current Sensor
  ECMOflow : Scope
      settings: ActiveDisplayYMinimum=-1  ActiveDisplayYMaximum=1  DataLoggingVariableName=ScopeData4
  PS-Simulink Converter6 : nesl_utility/PS-Simulink Converter  PhysicalDomain=network_engine_domain  SubClassName=ps_output  LeftPortType=input  RightPortType=output  PseudoPeriodic=off  Frequencies=[]  VectorFormat=1-D array  Unit=inherit  AffineConversion=on
  Out : PMIOPort  Side=Left
  In : PMIOPort  Port=2  Side=Right
  F90_ECMOFlowOut : Outport
  wires:
  PS-Simulink Converter6/1 -> ECMOflow/1, F90_ECMOFlowOut/1  "ECMOflow"
  connections:
  Current Sensor3/RConn1 -- PS-Simulink Converter6/LConn1
  Current Sensor3/LConn1 -- In/RConn1
  Current Sensor3/RConn2 -- Out/RConn1

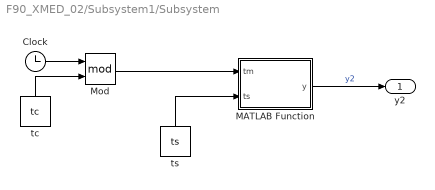
== system F90_XMED_02/Subsystem1/Subsystem ==
  Clock : Clock
  MATLAB Function : MATLAB Function  TreatAsAtomicUnit=on
  Mod : Math  Operator=mod
  tc : Constant  Value=tc
  ts : Constant  Value=ts
  y2 : Outport
  wires:
  Clock/1 -> Mod/1
  Mod/1 -> MATLAB Function/1(tm)
  MATLAB Function/1(y) -> y2/1  "y2"
  ts/1 -> MATLAB Function/2(ts)
  tc/1 -> Mod/2

== system F90_XMED_02/Subsystem12/Fixed ==
  R3 : fl_lib/Electrical/Electrical Elements/Resistor  R=R3 Ohm  i_specify=off  i_priority=None  i=0 A  i_nominal_specify=off  i_nominal_value=1  i_nominal_unit=A  v_specify=off  v_priority=None  v=0 V  v_nominal_specify=off  v_nominal_value=1  v_nominal_unit=V
  Conn1 : PMIOPort  Side=Left
  Conn2 : PMIOPort  Port=2  Side=Right
  connections:
  R3/RConn1 -- Conn2/RConn1
  R3/LConn1 -- Conn1/RConn1

== system F90_XMED_02/Subsystem12/Variable ==
  Signal Editor : SignalEditorBlockLib/Signal Editor  FileName=R3_Values.mat  ActiveScenario=Scenario  ActiveSignal=Signal 1  IsBus=off  OutputBusObjectStr=Bus: BusObject  SampleTime=0  Interpolate=off  ZeroCross=off  OutputAfterFinalValue=Holding final value  Unit=inherit  PreserveSignalName=on  ApplySigPropsToAllScenarios=on  ApplySigPropsToAllSignals=off  SignalPropertySource=Dialog parameters
  Simulink-PS Converter : nesl_utility/Simulink-PS Converter  PhysicalDomain=network_engine_domain  SubClassName=ps_input  LeftPortType=input  RightPortType=output  PseudoPeriodic=off  Frequencies=[]  NoiseDistribution=none  NoiseParameters=[]  Unit=1  AffineConversion=off  FilteringAndDerivatives=provide  SimscapeFilterOrder=1  InputFilterTimeConstant=0.001  UdotUserProvided=0
  Variable Resistor : fl_lib/Electrical/Electrical Elements/Variable Resistor  Rmin=0 Ohm  i_specify=off  i_priority=None  i=0 A  i_nominal_specify=off  i_nominal_unit=A  i_nominal_value=1  v_specify=off  v_priority=None  v=0 V  v_nominal_specify=off  v_nominal_unit=V  v_nominal_value=1
  Conn1 : PMIOPort  Side=Left
  Conn2 : PMIOPort  Port=2  Side=Right
  wires:
  Signal Editor/1 -> Simulink-PS Converter/1  "R3_ohm"
  connections:
  Variable Resistor/LConn1 -- Simulink-PS Converter/RConn1
  Variable Resistor/RConn1 -- Conn2/RConn1
  Variable Resistor/LConn2 -- Conn1/RConn1

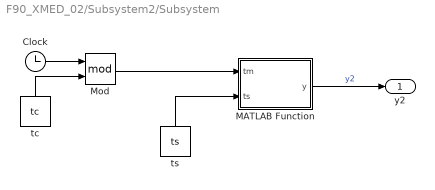
== system F90_XMED_02/Subsystem2/Subsystem ==
  Clock : Clock
  MATLAB Function : MATLAB Function  TreatAsAtomicUnit=on
  Mod : Math  Operator=mod
  tc : Constant  Value=tc
  ts : Constant  Value=ts
  y2 : Outport
  wires:
  Clock/1 -> Mod/1
  Mod/1 -> MATLAB Function/1(tm)
  MATLAB Function/1(y) -> y2/1  "y2"
  ts/1 -> MATLAB Function/2(ts)
  tc/1 -> Mod/2

== matlab function F90_XMED_02/Subsystem1/Subsystem/MATLAB Function ==
  data: tm input; y output; ts input
function y = fcn(tm, ts)

if(tm< ts)
    y = (1-cos(2*pi*tm/ts)) * 0.5;
else
    y = 0;
end

== matlab function F90_XMED_02/Subsystem2/Subsystem/MATLAB Function ==
  data: tm input; y output; ts input
function y = fcn(tm, ts)

if(tm< ts)
    y = (1-cos(2*pi*tm/ts)) * 0.5;
else
    y = 0;
end

== stateflow chart F90_XMED_02/Heart Phase Detector/Chart ==
  state HR_calc [parallel]
    settings: executionOrder=1
    state Init
      OffTime = 0;
      HR = 90;
    state On
      ex:
      %ONtime = elapsed(sec);
      ONtime = max(1/HR*0.2,elapsed(sec));
      HR = 0.5*HR + 0.5*60/( OffTime + ONtime);
      HR = min(220,HR);
      HR = max(50,HR);
      HR = Puls; % Override with set Pulse
    state Off
      du:
      OffTime = elapsed(sec);
    (default) -> Init
    Init -> HR_calc.On
    Off -> HR_calc.On : [ContractionTrue == true]
    HR_calc.On -> Off : [ContractionTrue == false]
  state CalcOutput [parallel]
    settings: executionOrder=2
    state On
      du:
      ContOut = true;
    state HRlessThan140
      du:
      ContOut = false;
    state HRMoreThan150
      % Inhibit true #1
      du:
      ContOut = false;
    state HRmoreThan140lessThan150
      % Inhibit true #1
      en:
      ContOut = false;
    state LastFalse
      ContOut = false;
    state False
      ContOut = false;
    state ThirdInhabitedTrue
      % Inhibit true #2
      ContOut = false;
    (default) -> CalcOutput.On
    HRlessThan140 -> CalcOutput.On [order 1] : [ContractionTrue == true & HR <140]
    HRlessThan140 -> HRMoreThan150 [order 3] : [ContractionTrue== true] % HR >= 150
    CalcOutput.On -> HRlessThan140 : [ContractionTrue==false]
    LastFalse -> CalcOutput.On : [ContractionTrue==true]
    HRlessThan140 -> HRmoreThan140lessThan150 [order 2] : [ContractionTrue == true  & true & HR < 150]
    HRmoreThan140lessThan150 -> LastFalse : [ContractionTrue == false ]
    HRMoreThan150 -> False : [ContractionTrue == false]
    ThirdInhabitedTrue -> LastFalse : [ContractionTrue==false]
    False -> ThirdInhabitedTrue : [ContractionTrue == true]
  data: ContractionTrue input; ContOut output; ONtime local; OffTime local; HR output; Puls input

== stateflow chart F90_XMED_02/Heart Phase Detector/Chart1 ==
  state Contracton
    du:
    MaxP = max(Pressure,MaxP);
    ContractionTrue = true;
    PressureOut = Pressure;
    MeanP = Pressure/1000+...
    999*MeanP/1000;
    LastP = Pressure;
  state Hold
    du:
    MaxP = max(Pressure,MaxP);
    ContractionTrue = true;
    PressureOut = Pressure;
    MeanP = Pressure/1000+...
    999*MeanP/1000;
    LastP = Pressure;
  state Init
    en:
    MaxP=Pressure;
    MinP = Pressure;
    MeanP = 50;
    LastP = Pressure;
  state NoContraction
    state NoContractionHold
      du:
      MinP = min(Pressure,MinP);
      ContractionTrue = false;
      PressureOut = 0;
      MeanP = Pressure/1000+...
      999*MeanP/1000;
      LastP = Pressure;
    state NoContraction
      du:
      MinP = min(Pressure,MinP);
      ContractionTrue = false;
      PressureOut = 0;
      MeanP = Pressure/1000+...
      999*MeanP/1000;
      LastP = Pressure;
    NoContractionHold -> NoContraction.NoContraction [order 2] : [LastP > Pressure]
    NoContraction.NoContraction -> NoContractionHold : [LastP<Pressure]
  (default) -> Init
  Init -> Contracton
  Contracton -> Hold : [LastP > Pressure]
  Hold -> Contracton [order 2] : [LastP<Pressure]
  Hold -> NoContraction.NoContraction [order 1] : after(WaitTime,sec){MaxP = Pressure;}
  NoContractionHold -> Contracton [order 1] : [after(WaitTime,sec) & Pressure < MeanP]{MinP = Pressure;}
  data: Pressure input; PressureOut output; ContractionTrue output; MaxP output; MinP output; MeanP output; LastP local; WaitTime input
